simulink model "p7_s"  (R2026a)
settings: Solver=VariableStepAuto
InitFcn:
  | Ra = 2;
  | Kt = 0.01;
  | b = 0.0012;
  | La = 0.023;
  | Ke = 0.01;
  | J = 0.001;
  | Va = 1;
libraries: fl_lib x9, nesl_utility x2
settings Model: Creator=Lcham

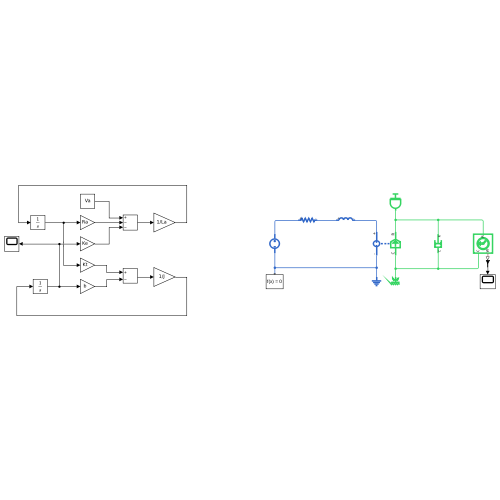
[thumbnail: Simulink's stored preview of the top-level diagram]
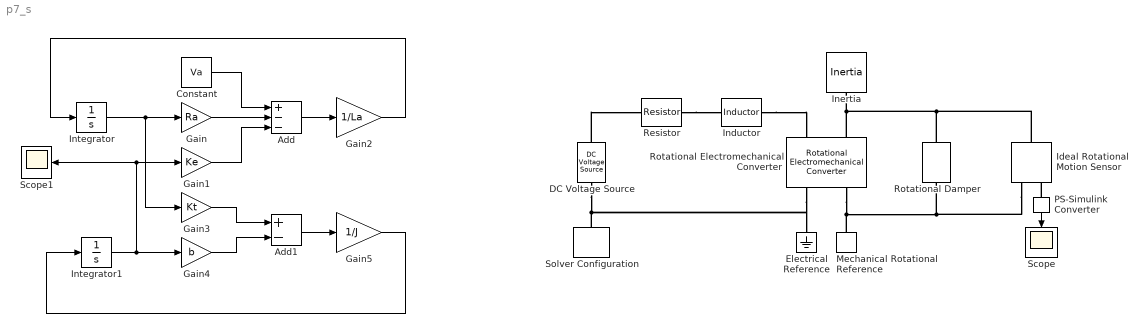
== system p7_s ==
  Add : Sum  Inputs=+--
  Add1 : Sum  Inputs=+-
  Constant : Constant  Value=Va
  DC Voltage Source : fl_lib/Electrical/Electrical Sources/DC Voltage Source  v0=Va V
  Electrical Reference : fl_lib/Electrical/Electrical Elements/Electrical Reference
  Gain : Gain  Gain=Ra
  Gain1 : Gain  Gain=Ke
  Gain2 : Gain  Gain=1/La
  Gain3 : Gain  Gain=Kt
  Gain4 : Gain  Gain=b
  Gain5 : Gain  Gain=1/J
  Ideal Rotational Motion Sensor : fl_lib/Mechanical/Mechanical Sensors/Ideal Rotational Motion Sensor  reference=foundation.enum.MeasurementReference.difference  acceleration_port=false  velocity_port=true  position_port=false  wrap_angle=false  offset=0 rad
  Inductor : fl_lib/Electrical/Electrical Elements/Inductor  l=.023 H  r=0 Ohm  g=1e-9 1/Ohm  i_specify=off  i_priority=None  i=0 A  i_nominal_specify=off  i_nominal_value=1  i_nominal_unit=A  v_specify=off  v_priority=None  v=0 V  v_nominal_specify=off  v_nominal_value=1  v_nominal_unit=V  i_L_specify=off  i_L_priority=High  i_L=0 A  i_L_nominal_specify=off  i_L_nominal_value=1  i_L_nominal_unit=A
  Inertia : fl_lib/Mechanical/Rotational Elements/Inertia  inertia=.001 kg*m^2  num_ports=foundation.enum.numPorts2.one  w_specify=off  w_priority=High  w=0 rad/s  w_nominal_specify=off  w_nominal_value=1  w_nominal_unit=rad/s  t_specify=off  t_priority=None  t=0 N*m  t_nominal_specify=off  t_nominal_value=1  t_nominal_unit=N*m
  Integrator : Integrator
  Integrator1 : Integrator
  Mechanical Rotational Reference : fl_lib/Mechanical/Rotational Elements/Mechanical Rotational Reference
  PS-Simulink Converter : nesl_utility/PS-Simulink Converter  PhysicalDomain=network_engine_domain  SubClassName=ps_output  LeftPortType=input  RightPortType=output  PseudoPeriodic=off  Frequencies=[]  VectorFormat=inherit  Unit=inherit  AffineConversion=off
  Resistor : fl_lib/Electrical/Electrical Elements/Resistor  R=2 Ohm  i_specify=off  i_priority=None  i=0 A  i_nominal_specify=off  i_nominal_value=1  i_nominal_unit=A  v_specify=off  v_priority=None  v=0 V  v_nominal_specify=off  v_nominal_value=1  v_nominal_unit=V
  Rotational Electromechanical Converter : fl_lib/Electrical/Electrical Elements/Rotational Electromechanical Converter  K=.01 V*s/rad  i_specify=off  i_priority=None  i=0 A  i_nominal_specify=off  i_nominal_value=1  i_nominal_unit=A  v_specify=off  v_priority=None  v=0 V  v_nominal_specify=off  v_nominal_value=1  v_nominal_unit=V  t_specify=off  t_priority=None  t=0 N*m  t_nominal_specify=off  t_nominal_value=1  t_nominal_unit=N*m  w_specify=off  w_priority=None  w=0 rad/s  w_nominal_specify=off  w_nominal_value=1  w_nominal_unit=rad/s
  Rotational Damper : fl_lib/Mechanical/Rotational Elements/Rotational Damper  D=.0012 N*m*s/rad  w_specify=off  w_priority=None  w=0 rad/s  w_nominal_specify=off  w_nominal_value=1  w_nominal_unit=rad/s  t_specify=off  t_priority=None  t=0 N*m  t_nominal_specify=off  t_nominal_value=1  t_nominal_unit=N*m
  Scope : Scope
      settings: ActiveDisplayYMinimum=-0.500004947269158  ActiveDisplayYMaximum=4.5000445254224228
  Scope1 : Scope
      settings: ActiveDisplayYMinimum=-0.50000494729003631  ActiveDisplayYMaximum=4.5000445256103276
  Solver Configuration : nesl_utility/Solver Configuration  PhysicalDomain=network_engine_domain  SubClassName=solver  LeftPortType=input  RightPortType=generic  Tones=[]  Harmonics=[]  SimulateNoise=off  Profile=off  UseLocalSampling=off  EnableSwitchedLinearOptims=on  FrequencyDomain=off  UseCCode=off  RelTol=0.001  AbsTol=0.001  MinStep=1e-09  ToWorkspace=off  RevertToSquareIcSolve=off  NumHomotopyIterations=100  PhasorMode=off  PhasorModeNumHarmonics=1  ConsistencySolver=NEWTON_XTOL_AFTER_FTOL  CanonicalOrdering=CANONICAL  OptimizeIntermediates=OPTIMIZED  IndexReductionMethod=DerivativeReplacement  DoDC=off  ResidualTolerance=1e-09  ConsistencyTolSource=GLOBAL  ConsistencyAbsTol=0.001  ConsistencyRelTol=0.001  ConsistencyTolFactor=0.001  UseLocalSolver=off  LocalSolverChoice=NE_BACKWARD_EULER_ADVANCER  ResolveIndetEquations=on  FunctionEvalNumThread=1  LocalSolverSampleTime=0.001  DoFixedCost=off  MaxNonlinIter=3  MaxModeIter=2  ComputeImpulses=off  ImpulseIterations=2  LinearAlgebra=auto  LinearAlgebraNumThread=0  EquationFormulation=NE_TIME_EF  DelaysMemoryBudget=1024  AutomaticFiltering=on  FilteringTimeConstant=0.001  PartitionStorageMethod=AS_NEEDED  PartitionMemoryBudget=1024  PartitionMethod=ROBUST  MultibodyUseLocalSolver=off  MultibodyLocalSolverChoice=ODE1  MultibodyLocalSolverSampleTime=0.001
  wires:
  PS-Simulink Converter/1 -> Scope/1
  Integrator/1 -> Gain3/1, Gain/1
  Integrator1/1 -> Scope1/1, Gain1/1, Gain4/1
  Gain/1 -> Add/2
  Gain1/1 -> Add/3
  Constant/1 -> Add/1
  Add/1 -> Gain2/1
  Gain2/1 -> Integrator/1
  Gain3/1 -> Add1/1
  Gain4/1 -> Add1/2
  Add1/1 -> Gain5/1
  Gain5/1 -> Integrator1/1
  connections:
  Solver Configuration/RConn1 -- Rotational Electromechanical Converter/RConn1 -- Electrical Reference/LConn1 -- DC Voltage Source/RConn1
  Mechanical Rotational Reference/LConn1 -- Rotational Electromechanical Converter/RConn2 -- Rotational Damper/RConn1 -- Ideal Rotational Motion Sensor/RConn1
  Rotational Damper/LConn1 -- Rotational Electromechanical Converter/LConn2 -- Inertia/LConn1 -- Ideal Rotational Motion Sensor/LConn1
  PS-Simulink Converter/LConn1 -- Ideal Rotational Motion Sensor/RConn2
  Resistor/RConn1 -- Inductor/LConn1
  DC Voltage Source/LConn1 -- Resistor/LConn1
  Inductor/RConn1 -- Rotational Electromechanical Converter/LConn1
